simulink model "six_pulse_dstack_based_rectifier"  (R2026a)
settings: Solver=ode23tb  StopTime=simlength  FixedStep=Ts  MaxStep=Tc  EnableMultiTasking=on
values from neighbouring files (symbols this model uses):
  Csnubber = 0.1e-6    (= 1e-07)    [init_model.m]
  LFu_dc = 1.2e-3    (= 0.0012)    [init_model.m]
  Rgrading = 2.4e6    (= 2400000)    [init_model.m]
  RLFu_dc = 2e-4    (= 0.0002)    [init_model.m]
  Rsnubber = 1000    [init_model.m]
  Tc = Tcontrol_rect/4000    (= 5e-08)    [init_model.m]
  Tcontrol_rect = tPWM_RECT    (= 0.0002)    [init_model.m]
  Vnom_ac_adc = 400/sqrt(3)*sqrt(2)    [init_model.m]
  w_grid = f_grid*2*pi    (= 314.159265359)    [init_model.m]
undefined symbols (not defined in the file or in its folder): magnitude, rms
libraries: fl_lib x179, nesl_utility x129, diode_rr_lib x36, ee_lib x2
(part 4 of 5)

== system six_pulse_dstack_based_rectifier/six_pulse rectifier/BR2/ssc_diode_rr_bridge/D4/D11/D11 ==
  Capacitor : fl_lib/Electrical/Electrical Elements/Capacitor  c=Csnubber_m F  r=Rsnubber_m Ohm  g=0 1/Ohm  i_specify=off  i_priority=None  i=0 A  i_nominal_specify=off  i_nominal_value=1  i_nominal_unit=A  v_specify=off  v_priority=None  v=0 V  v_nominal_specify=off  v_nominal_value=1  v_nominal_unit=V  vc_specify=off  vc_priority=High  vc=0 V  vc_nominal_specify=off  vc_nominal_value=1  vc_nominal_unit=V
  Current Sensor : fl_lib/Electrical/Electrical Sensors/Current Sensor
  Current Sensor1 : fl_lib/Electrical/Electrical Sensors/Current Sensor
  PS-Simulink Converter : nesl_utility/PS-Simulink Converter  PhysicalDomain=network_engine_domain  SubClassName=ps_output  LeftPortType=input  RightPortType=output  PseudoPeriodic=off  Frequencies=[]  VectorFormat=1-D array  Unit=A  AffineConversion=off
  PS-Simulink Converter1 : nesl_utility/PS-Simulink Converter  PhysicalDomain=network_engine_domain  SubClassName=ps_output  LeftPortType=input  RightPortType=output  PseudoPeriodic=off  Frequencies=[]  VectorFormat=1-D array  Unit=V  AffineConversion=off
  PS-Simulink Converter2 : nesl_utility/PS-Simulink Converter  PhysicalDomain=network_engine_domain  SubClassName=ps_output  LeftPortType=input  RightPortType=output  PseudoPeriodic=off  Frequencies=[]  VectorFormat=1-D array  Unit=A  AffineConversion=off
  RR Diode (Lauritzen-Ma) : diode_rr_lib/RR Diode (Lauritzen-Ma)  Is=5e-9 A  N=2  Vt=26e-3 V  tau=350e-9 s  TM=60e-9 s  Rs=0.5e-3 Ohm  Cj0=10e-9 F  Vjp=0.7 V  mg=0.5  FC=0.5  dsm=10e-3 V  i_specify=off  i_priority=None  i=0 A  i_nominal_specify=off  i_nominal_value=1  i_nominal_unit=A  v_specify=off  v_priority=None  v=0 V  v_nominal_specify=off  v_nominal_value=1  v_nominal_unit=V  vj_specify=off  vj_priority=None  vj=0 V  vj_nominal_specify=off  vj_nominal_value=1  vj_nominal_unit=V  qE_specify=off  qE_priority=None  qE=0 C  qE_nominal_specify=off  qE_nominal_value=1e-4  qE_nominal_unit=C  qM_specify=off  qM_priority=High  qM=0 C  qM_nominal_specify=off  qM_nominal_value=1e-4  qM_nominal_unit=C  qj_specify=off  qj_priority=None  qj=0 C  qj_nominal_specify=off  qj_nominal_value=1e-5  qj_nominal_unit=C
  Voltage Sensor : fl_lib/Electrical/Electrical Sensors/Voltage Sensor
  K : PMIOPort  Side=Left
  A : PMIOPort  Port=2  Side=Right
  tag scope: D11_Id=scoped, D11_Ud=scoped, RC11_Id=scoped
  wires:
  PS-Simulink Converter/1 -> [D11_Id]
  PS-Simulink Converter2/1 -> [RC11_Id]
  PS-Simulink Converter1/1 -> [D11_Ud]
  connections:
  Voltage Sensor/RConn2 -- K/RConn1 -- Capacitor/LConn1 -- RR Diode (Lauritzen-Ma)/RConn1
  PS-Simulink Converter1/LConn1 -- Voltage Sensor/RConn1
  PS-Simulink Converter/LConn1 -- Current Sensor/RConn1
  Current Sensor1/RConn2 -- Capacitor/RConn1
  Voltage Sensor/LConn1 -- Current Sensor1/LConn1 -- Current Sensor/RConn2 -- RR Diode (Lauritzen-Ma)/LConn1
  PS-Simulink Converter2/LConn1 -- Current Sensor1/RConn1
  A/RConn1 -- Current Sensor/LConn1

== system six_pulse_dstack_based_rectifier/six_pulse rectifier/BR2/ssc_diode_rr_bridge/D4/D12/D12 ==
  Capacitor : fl_lib/Electrical/Electrical Elements/Capacitor  c=Csnubber_m F  r=Rsnubber_m Ohm  g=0 1/Ohm  i_specify=off  i_priority=None  i=0 A  i_nominal_specify=off  i_nominal_value=1  i_nominal_unit=A  v_specify=off  v_priority=None  v=0 V  v_nominal_specify=off  v_nominal_value=1  v_nominal_unit=V  vc_specify=off  vc_priority=High  vc=0 V  vc_nominal_specify=off  vc_nominal_value=1  vc_nominal_unit=V
  Current Sensor : fl_lib/Electrical/Electrical Sensors/Current Sensor
  Current Sensor1 : fl_lib/Electrical/Electrical Sensors/Current Sensor
  PS-Simulink Converter : nesl_utility/PS-Simulink Converter  PhysicalDomain=network_engine_domain  SubClassName=ps_output  LeftPortType=input  RightPortType=output  PseudoPeriodic=off  Frequencies=[]  VectorFormat=1-D array  Unit=A  AffineConversion=off
  PS-Simulink Converter1 : nesl_utility/PS-Simulink Converter  PhysicalDomain=network_engine_domain  SubClassName=ps_output  LeftPortType=input  RightPortType=output  PseudoPeriodic=off  Frequencies=[]  VectorFormat=1-D array  Unit=V  AffineConversion=off
  PS-Simulink Converter2 : nesl_utility/PS-Simulink Converter  PhysicalDomain=network_engine_domain  SubClassName=ps_output  LeftPortType=input  RightPortType=output  PseudoPeriodic=off  Frequencies=[]  VectorFormat=1-D array  Unit=A  AffineConversion=off
  RR Diode (Lauritzen-Ma) : diode_rr_lib/RR Diode (Lauritzen-Ma)  Is=5e-9 A  N=2  Vt=26e-3 V  tau=350e-9 s  TM=60e-9 s  Rs=0.5e-3 Ohm  Cj0=10e-9 F  Vjp=0.7 V  mg=0.5  FC=0.5  dsm=10e-3 V  i_specify=off  i_priority=None  i=0 A  i_nominal_specify=off  i_nominal_value=1  i_nominal_unit=A  v_specify=off  v_priority=None  v=0 V  v_nominal_specify=off  v_nominal_value=1  v_nominal_unit=V  vj_specify=off  vj_priority=None  vj=0 V  vj_nominal_specify=off  vj_nominal_value=1  vj_nominal_unit=V  qE_specify=off  qE_priority=None  qE=0 C  qE_nominal_specify=off  qE_nominal_value=1e-4  qE_nominal_unit=C  qM_specify=off  qM_priority=High  qM=0 C  qM_nominal_specify=off  qM_nominal_value=1e-4  qM_nominal_unit=C  qj_specify=off  qj_priority=None  qj=0 C  qj_nominal_specify=off  qj_nominal_value=1e-5  qj_nominal_unit=C
  Voltage Sensor : fl_lib/Electrical/Electrical Sensors/Voltage Sensor
  K : PMIOPort  Side=Left
  A : PMIOPort  Port=2  Side=Right
  tag scope: D12_Id=scoped, D12_Ud=scoped, RC12_Id=scoped
  wires:
  PS-Simulink Converter1/1 -> [D12_Ud]
  PS-Simulink Converter2/1 -> [RC12_Id]
  PS-Simulink Converter/1 -> [D12_Id]
  connections:
  A/RConn1 -- Current Sensor/LConn1
  PS-Simulink Converter2/LConn1 -- Current Sensor1/RConn1
  RR Diode (Lauritzen-Ma)/LConn1 -- Current Sensor/RConn2 -- Current Sensor1/LConn1 -- Voltage Sensor/LConn1
  Current Sensor1/RConn2 -- Capacitor/RConn1
  PS-Simulink Converter/LConn1 -- Current Sensor/RConn1
  PS-Simulink Converter1/LConn1 -- Voltage Sensor/RConn1
  RR Diode (Lauritzen-Ma)/RConn1 -- Capacitor/LConn1 -- Voltage Sensor/RConn2 -- K/RConn1

== system six_pulse_dstack_based_rectifier/six_pulse rectifier/BR2/ssc_diode_rr_bridge/D4/D13/D13 ==
  Capacitor : fl_lib/Electrical/Electrical Elements/Capacitor  c=Csnubber_m F  r=Rsnubber_m Ohm  g=0 1/Ohm  i_specify=off  i_priority=None  i=0 A  i_nominal_specify=off  i_nominal_value=1  i_nominal_unit=A  v_specify=off  v_priority=None  v=0 V  v_nominal_specify=off  v_nominal_value=1  v_nominal_unit=V  vc_specify=off  vc_priority=High  vc=0 V  vc_nominal_specify=off  vc_nominal_value=1  vc_nominal_unit=V
  Current Sensor : fl_lib/Electrical/Electrical Sensors/Current Sensor
  Current Sensor1 : fl_lib/Electrical/Electrical Sensors/Current Sensor
  PS-Simulink Converter : nesl_utility/PS-Simulink Converter  PhysicalDomain=network_engine_domain  SubClassName=ps_output  LeftPortType=input  RightPortType=output  PseudoPeriodic=off  Frequencies=[]  VectorFormat=1-D array  Unit=A  AffineConversion=off
  PS-Simulink Converter1 : nesl_utility/PS-Simulink Converter  PhysicalDomain=network_engine_domain  SubClassName=ps_output  LeftPortType=input  RightPortType=output  PseudoPeriodic=off  Frequencies=[]  VectorFormat=1-D array  Unit=V  AffineConversion=off
  PS-Simulink Converter2 : nesl_utility/PS-Simulink Converter  PhysicalDomain=network_engine_domain  SubClassName=ps_output  LeftPortType=input  RightPortType=output  PseudoPeriodic=off  Frequencies=[]  VectorFormat=1-D array  Unit=A  AffineConversion=off
  RR Diode (Lauritzen-Ma) : diode_rr_lib/RR Diode (Lauritzen-Ma)  Is=5e-9 A  N=2  Vt=26e-3 V  tau=350e-9 s  TM=60e-9 s  Rs=0.5e-3 Ohm  Cj0=10e-9 F  Vjp=0.7 V  mg=0.5  FC=0.5  dsm=10e-3 V  i_specify=off  i_priority=None  i=0 A  i_nominal_specify=off  i_nominal_value=1  i_nominal_unit=A  v_specify=off  v_priority=None  v=0 V  v_nominal_specify=off  v_nominal_value=1  v_nominal_unit=V  vj_specify=off  vj_priority=None  vj=0 V  vj_nominal_specify=off  vj_nominal_value=1  vj_nominal_unit=V  qE_specify=off  qE_priority=None  qE=0 C  qE_nominal_specify=off  qE_nominal_value=1e-4  qE_nominal_unit=C  qM_specify=off  qM_priority=High  qM=0 C  qM_nominal_specify=off  qM_nominal_value=1e-4  qM_nominal_unit=C  qj_specify=off  qj_priority=None  qj=0 C  qj_nominal_specify=off  qj_nominal_value=1e-5  qj_nominal_unit=C
  Voltage Sensor : fl_lib/Electrical/Electrical Sensors/Voltage Sensor
  K : PMIOPort  Side=Left
  A : PMIOPort  Port=2  Side=Right
  tag scope: D13_Id=scoped, D13_Ud=scoped, RC13_Id=scoped
  wires:
  PS-Simulink Converter/1 -> [D13_Id]
  PS-Simulink Converter2/1 -> [RC13_Id]
  PS-Simulink Converter1/1 -> [D13_Ud]
  connections:
  K/RConn1 -- Voltage Sensor/RConn2 -- Capacitor/LConn1 -- RR Diode (Lauritzen-Ma)/RConn1
  PS-Simulink Converter1/LConn1 -- Voltage Sensor/RConn1
  PS-Simulink Converter/LConn1 -- Current Sensor/RConn1
  Current Sensor1/RConn2 -- Capacitor/RConn1
  Voltage Sensor/LConn1 -- Current Sensor1/LConn1 -- Current Sensor/RConn2 -- RR Diode (Lauritzen-Ma)/LConn1
  PS-Simulink Converter2/LConn1 -- Current Sensor1/RConn1
  A/RConn1 -- Current Sensor/LConn1

== system six_pulse_dstack_based_rectifier/six_pulse rectifier/BR2/ssc_diode_rr_bridge/D4/D14/D14 ==
  Capacitor : fl_lib/Electrical/Electrical Elements/Capacitor  c=Csnubber_m F  r=Rsnubber_m Ohm  g=0 1/Ohm  i_specify=off  i_priority=None  i=0 A  i_nominal_specify=off  i_nominal_value=1  i_nominal_unit=A  v_specify=off  v_priority=None  v=0 V  v_nominal_specify=off  v_nominal_value=1  v_nominal_unit=V  vc_specify=off  vc_priority=High  vc=0 V  vc_nominal_specify=off  vc_nominal_value=1  vc_nominal_unit=V
  Current Sensor : fl_lib/Electrical/Electrical Sensors/Current Sensor
  Current Sensor1 : fl_lib/Electrical/Electrical Sensors/Current Sensor
  PS-Simulink Converter : nesl_utility/PS-Simulink Converter  PhysicalDomain=network_engine_domain  SubClassName=ps_output  LeftPortType=input  RightPortType=output  PseudoPeriodic=off  Frequencies=[]  VectorFormat=1-D array  Unit=A  AffineConversion=off
  PS-Simulink Converter1 : nesl_utility/PS-Simulink Converter  PhysicalDomain=network_engine_domain  SubClassName=ps_output  LeftPortType=input  RightPortType=output  PseudoPeriodic=off  Frequencies=[]  VectorFormat=1-D array  Unit=V  AffineConversion=off
  PS-Simulink Converter2 : nesl_utility/PS-Simulink Converter  PhysicalDomain=network_engine_domain  SubClassName=ps_output  LeftPortType=input  RightPortType=output  PseudoPeriodic=off  Frequencies=[]  VectorFormat=1-D array  Unit=A  AffineConversion=off
  RR Diode (Lauritzen-Ma) : diode_rr_lib/RR Diode (Lauritzen-Ma)  Is=5e-9 A  N=2  Vt=26e-3 V  tau=350e-9 s  TM=60e-9 s  Rs=0.5e-3 Ohm  Cj0=10e-9 F  Vjp=0.7 V  mg=0.5  FC=0.5  dsm=10e-3 V  i_specify=off  i_priority=None  i=0 A  i_nominal_specify=off  i_nominal_value=1  i_nominal_unit=A  v_specify=off  v_priority=None  v=0 V  v_nominal_specify=off  v_nominal_value=1  v_nominal_unit=V  vj_specify=off  vj_priority=None  vj=0 V  vj_nominal_specify=off  vj_nominal_value=1  vj_nominal_unit=V  qE_specify=off  qE_priority=None  qE=0 C  qE_nominal_specify=off  qE_nominal_value=1e-4  qE_nominal_unit=C  qM_specify=off  qM_priority=High  qM=0 C  qM_nominal_specify=off  qM_nominal_value=1e-4  qM_nominal_unit=C  qj_specify=off  qj_priority=None  qj=0 C  qj_nominal_specify=off  qj_nominal_value=1e-5  qj_nominal_unit=C
  Voltage Sensor : fl_lib/Electrical/Electrical Sensors/Voltage Sensor
  K : PMIOPort  Side=Left
  A : PMIOPort  Port=2  Side=Right
  tag scope: D14_Id=scoped, D14_Ud=scoped, RC14_Id=scoped
  wires:
  PS-Simulink Converter1/1 -> [D14_Ud]
  PS-Simulink Converter2/1 -> [RC14_Id]
  PS-Simulink Converter/1 -> [D14_Id]
  connections:
  A/RConn1 -- Current Sensor/LConn1
  PS-Simulink Converter2/LConn1 -- Current Sensor1/RConn1
  RR Diode (Lauritzen-Ma)/LConn1 -- Current Sensor/RConn2 -- Current Sensor1/LConn1 -- Voltage Sensor/LConn1
  Current Sensor1/RConn2 -- Capacitor/RConn1
  PS-Simulink Converter/LConn1 -- Current Sensor/RConn1
  PS-Simulink Converter1/LConn1 -- Voltage Sensor/RConn1
  RR Diode (Lauritzen-Ma)/RConn1 -- Capacitor/LConn1 -- Voltage Sensor/RConn2 -- K/RConn1

== system six_pulse_dstack_based_rectifier/six_pulse rectifier/BR2/ssc_diode_rr_bridge/D4/D15/D15 ==
  Capacitor : fl_lib/Electrical/Electrical Elements/Capacitor  c=Csnubber_m F  r=Rsnubber_m Ohm  g=0 1/Ohm  i_specify=off  i_priority=None  i=0 A  i_nominal_specify=off  i_nominal_value=1  i_nominal_unit=A  v_specify=off  v_priority=None  v=0 V  v_nominal_specify=off  v_nominal_value=1  v_nominal_unit=V  vc_specify=off  vc_priority=High  vc=0 V  vc_nominal_specify=off  vc_nominal_value=1  vc_nominal_unit=V
  Current Sensor : fl_lib/Electrical/Electrical Sensors/Current Sensor
  Current Sensor1 : fl_lib/Electrical/Electrical Sensors/Current Sensor
  PS-Simulink Converter : nesl_utility/PS-Simulink Converter  PhysicalDomain=network_engine_domain  SubClassName=ps_output  LeftPortType=input  RightPortType=output  PseudoPeriodic=off  Frequencies=[]  VectorFormat=1-D array  Unit=A  AffineConversion=off
  PS-Simulink Converter1 : nesl_utility/PS-Simulink Converter  PhysicalDomain=network_engine_domain  SubClassName=ps_output  LeftPortType=input  RightPortType=output  PseudoPeriodic=off  Frequencies=[]  VectorFormat=1-D array  Unit=V  AffineConversion=off
  PS-Simulink Converter2 : nesl_utility/PS-Simulink Converter  PhysicalDomain=network_engine_domain  SubClassName=ps_output  LeftPortType=input  RightPortType=output  PseudoPeriodic=off  Frequencies=[]  VectorFormat=1-D array  Unit=A  AffineConversion=off
  RR Diode (Lauritzen-Ma) : diode_rr_lib/RR Diode (Lauritzen-Ma)  Is=5e-9 A  N=2  Vt=26e-3 V  tau=350e-9 s  TM=60e-9 s  Rs=0.5e-3 Ohm  Cj0=10e-9 F  Vjp=0.7 V  mg=0.5  FC=0.5  dsm=10e-3 V  i_specify=off  i_priority=None  i=0 A  i_nominal_specify=off  i_nominal_value=1  i_nominal_unit=A  v_specify=off  v_priority=None  v=0 V  v_nominal_specify=off  v_nominal_value=1  v_nominal_unit=V  vj_specify=off  vj_priority=None  vj=0 V  vj_nominal_specify=off  vj_nominal_value=1  vj_nominal_unit=V  qE_specify=off  qE_priority=None  qE=0 C  qE_nominal_specify=off  qE_nominal_value=1e-4  qE_nominal_unit=C  qM_specify=off  qM_priority=High  qM=0 C  qM_nominal_specify=off  qM_nominal_value=1e-4  qM_nominal_unit=C  qj_specify=off  qj_priority=None  qj=0 C  qj_nominal_specify=off  qj_nominal_value=1e-5  qj_nominal_unit=C
  Voltage Sensor : fl_lib/Electrical/Electrical Sensors/Voltage Sensor
  K : PMIOPort  Side=Left
  A : PMIOPort  Port=2  Side=Right
  tag scope: D15_Id=scoped, D15_Ud=scoped, RC15_Id=scoped
  wires:
  PS-Simulink Converter/1 -> [D15_Id]
  PS-Simulink Converter2/1 -> [RC15_Id]
  PS-Simulink Converter1/1 -> [D15_Ud]
  connections:
  K/RConn1 -- Voltage Sensor/RConn2 -- Capacitor/LConn1 -- RR Diode (Lauritzen-Ma)/RConn1
  PS-Simulink Converter1/LConn1 -- Voltage Sensor/RConn1
  PS-Simulink Converter/LConn1 -- Current Sensor/RConn1
  Current Sensor1/RConn2 -- Capacitor/RConn1
  Voltage Sensor/LConn1 -- Current Sensor1/LConn1 -- Current Sensor/RConn2 -- RR Diode (Lauritzen-Ma)/LConn1
  PS-Simulink Converter2/LConn1 -- Current Sensor1/RConn1
  A/RConn1 -- Current Sensor/LConn1

== system six_pulse_dstack_based_rectifier/six_pulse rectifier/BR2/ssc_diode_rr_bridge/D4/D16/D16 ==
  Capacitor : fl_lib/Electrical/Electrical Elements/Capacitor  c=Csnubber_m F  r=Rsnubber_m Ohm  g=0 1/Ohm  i_specify=off  i_priority=None  i=0 A  i_nominal_specify=off  i_nominal_value=1  i_nominal_unit=A  v_specify=off  v_priority=None  v=0 V  v_nominal_specify=off  v_nominal_value=1  v_nominal_unit=V  vc_specify=off  vc_priority=High  vc=0 V  vc_nominal_specify=off  vc_nominal_value=1  vc_nominal_unit=V
  Current Sensor : fl_lib/Electrical/Electrical Sensors/Current Sensor
  Current Sensor1 : fl_lib/Electrical/Electrical Sensors/Current Sensor
  PS-Simulink Converter : nesl_utility/PS-Simulink Converter  PhysicalDomain=network_engine_domain  SubClassName=ps_output  LeftPortType=input  RightPortType=output  PseudoPeriodic=off  Frequencies=[]  VectorFormat=1-D array  Unit=A  AffineConversion=off
  PS-Simulink Converter1 : nesl_utility/PS-Simulink Converter  PhysicalDomain=network_engine_domain  SubClassName=ps_output  LeftPortType=input  RightPortType=output  PseudoPeriodic=off  Frequencies=[]  VectorFormat=1-D array  Unit=V  AffineConversion=off
  PS-Simulink Converter2 : nesl_utility/PS-Simulink Converter  PhysicalDomain=network_engine_domain  SubClassName=ps_output  LeftPortType=input  RightPortType=output  PseudoPeriodic=off  Frequencies=[]  VectorFormat=1-D array  Unit=A  AffineConversion=off
  RR Diode (Lauritzen-Ma) : diode_rr_lib/RR Diode (Lauritzen-Ma)  Is=5e-9 A  N=2  Vt=26e-3 V  tau=350e-9 s  TM=60e-9 s  Rs=0.5e-3 Ohm  Cj0=10e-9 F  Vjp=0.7 V  mg=0.5  FC=0.5  dsm=10e-3 V  i_specify=off  i_priority=None  i=0 A  i_nominal_specify=off  i_nominal_value=1  i_nominal_unit=A  v_specify=off  v_priority=None  v=0 V  v_nominal_specify=off  v_nominal_value=1  v_nominal_unit=V  vj_specify=off  vj_priority=None  vj=0 V  vj_nominal_specify=off  vj_nominal_value=1  vj_nominal_unit=V  qE_specify=off  qE_priority=None  qE=0 C  qE_nominal_specify=off  qE_nominal_value=1e-4  qE_nominal_unit=C  qM_specify=off  qM_priority=High  qM=0 C  qM_nominal_specify=off  qM_nominal_value=1e-4  qM_nominal_unit=C  qj_specify=off  qj_priority=None  qj=0 C  qj_nominal_specify=off  qj_nominal_value=1e-5  qj_nominal_unit=C
  Voltage Sensor : fl_lib/Electrical/Electrical Sensors/Voltage Sensor
  K : PMIOPort  Side=Left
  A : PMIOPort  Port=2  Side=Right
  tag scope: D16_Id=scoped, D16_Ud=scoped, RC16_Id=scoped
  wires:
  PS-Simulink Converter1/1 -> [D16_Ud]
  PS-Simulink Converter2/1 -> [RC16_Id]
  PS-Simulink Converter/1 -> [D16_Id]
  connections:
  A/RConn1 -- Current Sensor/LConn1
  PS-Simulink Converter2/LConn1 -- Current Sensor1/RConn1
  RR Diode (Lauritzen-Ma)/LConn1 -- Current Sensor/RConn2 -- Current Sensor1/LConn1 -- Voltage Sensor/LConn1
  Current Sensor1/RConn2 -- Capacitor/RConn1
  PS-Simulink Converter/LConn1 -- Current Sensor/RConn1
  PS-Simulink Converter1/LConn1 -- Voltage Sensor/RConn1
  RR Diode (Lauritzen-Ma)/RConn1 -- Capacitor/LConn1 -- Voltage Sensor/RConn2 -- K/RConn1

== system six_pulse_dstack_based_rectifier/six_pulse rectifier/BR2/ssc_diode_rr_bridge/D5/D11/D11 ==
  Capacitor : fl_lib/Electrical/Electrical Elements/Capacitor  c=Csnubber_m F  r=Rsnubber_m Ohm  g=0 1/Ohm  i_specify=off  i_priority=None  i=0 A  i_nominal_specify=off  i_nominal_value=1  i_nominal_unit=A  v_specify=off  v_priority=None  v=0 V  v_nominal_specify=off  v_nominal_value=1  v_nominal_unit=V  vc_specify=off  vc_priority=High  vc=0 V  vc_nominal_specify=off  vc_nominal_value=1  vc_nominal_unit=V
  Current Sensor : fl_lib/Electrical/Electrical Sensors/Current Sensor
  Current Sensor1 : fl_lib/Electrical/Electrical Sensors/Current Sensor
  PS-Simulink Converter : nesl_utility/PS-Simulink Converter  PhysicalDomain=network_engine_domain  SubClassName=ps_output  LeftPortType=input  RightPortType=output  PseudoPeriodic=off  Frequencies=[]  VectorFormat=1-D array  Unit=A  AffineConversion=off
  PS-Simulink Converter1 : nesl_utility/PS-Simulink Converter  PhysicalDomain=network_engine_domain  SubClassName=ps_output  LeftPortType=input  RightPortType=output  PseudoPeriodic=off  Frequencies=[]  VectorFormat=1-D array  Unit=V  AffineConversion=off
  PS-Simulink Converter2 : nesl_utility/PS-Simulink Converter  PhysicalDomain=network_engine_domain  SubClassName=ps_output  LeftPortType=input  RightPortType=output  PseudoPeriodic=off  Frequencies=[]  VectorFormat=1-D array  Unit=A  AffineConversion=off
  RR Diode (Lauritzen-Ma) : diode_rr_lib/RR Diode (Lauritzen-Ma)  Is=5e-9 A  N=2  Vt=26e-3 V  tau=350e-9 s  TM=60e-9 s  Rs=0.5e-3 Ohm  Cj0=10e-9 F  Vjp=0.7 V  mg=0.5  FC=0.5  dsm=10e-3 V  i_specify=off  i_priority=None  i=0 A  i_nominal_specify=off  i_nominal_value=1  i_nominal_unit=A  v_specify=off  v_priority=None  v=0 V  v_nominal_specify=off  v_nominal_value=1  v_nominal_unit=V  vj_specify=off  vj_priority=None  vj=0 V  vj_nominal_specify=off  vj_nominal_value=1  vj_nominal_unit=V  qE_specify=off  qE_priority=None  qE=0 C  qE_nominal_specify=off  qE_nominal_value=1e-4  qE_nominal_unit=C  qM_specify=off  qM_priority=High  qM=0 C  qM_nominal_specify=off  qM_nominal_value=1e-4  qM_nominal_unit=C  qj_specify=off  qj_priority=None  qj=0 C  qj_nominal_specify=off  qj_nominal_value=1e-5  qj_nominal_unit=C
  Voltage Sensor : fl_lib/Electrical/Electrical Sensors/Voltage Sensor
  K : PMIOPort  Side=Left
  A : PMIOPort  Port=2  Side=Right
  tag scope: D11_Id=scoped, D11_Ud=scoped, RC11_Id=scoped
  wires:
  PS-Simulink Converter/1 -> [D11_Id]
  PS-Simulink Converter2/1 -> [RC11_Id]
  PS-Simulink Converter1/1 -> [D11_Ud]
  connections:
  Voltage Sensor/RConn2 -- K/RConn1 -- Capacitor/LConn1 -- RR Diode (Lauritzen-Ma)/RConn1
  PS-Simulink Converter1/LConn1 -- Voltage Sensor/RConn1
  PS-Simulink Converter/LConn1 -- Current Sensor/RConn1
  Current Sensor1/RConn2 -- Capacitor/RConn1
  Voltage Sensor/LConn1 -- Current Sensor1/LConn1 -- Current Sensor/RConn2 -- RR Diode (Lauritzen-Ma)/LConn1
  PS-Simulink Converter2/LConn1 -- Current Sensor1/RConn1
  A/RConn1 -- Current Sensor/LConn1

== system six_pulse_dstack_based_rectifier/six_pulse rectifier/BR2/ssc_diode_rr_bridge/D5/D12/D12 ==
  Capacitor : fl_lib/Electrical/Electrical Elements/Capacitor  c=Csnubber_m F  r=Rsnubber_m Ohm  g=0 1/Ohm  i_specify=off  i_priority=None  i=0 A  i_nominal_specify=off  i_nominal_value=1  i_nominal_unit=A  v_specify=off  v_priority=None  v=0 V  v_nominal_specify=off  v_nominal_value=1  v_nominal_unit=V  vc_specify=off  vc_priority=High  vc=0 V  vc_nominal_specify=off  vc_nominal_value=1  vc_nominal_unit=V
  Current Sensor : fl_lib/Electrical/Electrical Sensors/Current Sensor
  Current Sensor1 : fl_lib/Electrical/Electrical Sensors/Current Sensor
  PS-Simulink Converter : nesl_utility/PS-Simulink Converter  PhysicalDomain=network_engine_domain  SubClassName=ps_output  LeftPortType=input  RightPortType=output  PseudoPeriodic=off  Frequencies=[]  VectorFormat=1-D array  Unit=A  AffineConversion=off
  PS-Simulink Converter1 : nesl_utility/PS-Simulink Converter  PhysicalDomain=network_engine_domain  SubClassName=ps_output  LeftPortType=input  RightPortType=output  PseudoPeriodic=off  Frequencies=[]  VectorFormat=1-D array  Unit=V  AffineConversion=off
  PS-Simulink Converter2 : nesl_utility/PS-Simulink Converter  PhysicalDomain=network_engine_domain  SubClassName=ps_output  LeftPortType=input  RightPortType=output  PseudoPeriodic=off  Frequencies=[]  VectorFormat=1-D array  Unit=A  AffineConversion=off
  RR Diode (Lauritzen-Ma) : diode_rr_lib/RR Diode (Lauritzen-Ma)  Is=5e-9 A  N=2  Vt=26e-3 V  tau=350e-9 s  TM=60e-9 s  Rs=0.5e-3 Ohm  Cj0=10e-9 F  Vjp=0.7 V  mg=0.5  FC=0.5  dsm=10e-3 V  i_specify=off  i_priority=None  i=0 A  i_nominal_specify=off  i_nominal_value=1  i_nominal_unit=A  v_specify=off  v_priority=None  v=0 V  v_nominal_specify=off  v_nominal_value=1  v_nominal_unit=V  vj_specify=off  vj_priority=None  vj=0 V  vj_nominal_specify=off  vj_nominal_value=1  vj_nominal_unit=V  qE_specify=off  qE_priority=None  qE=0 C  qE_nominal_specify=off  qE_nominal_value=1e-4  qE_nominal_unit=C  qM_specify=off  qM_priority=High  qM=0 C  qM_nominal_specify=off  qM_nominal_value=1e-4  qM_nominal_unit=C  qj_specify=off  qj_priority=None  qj=0 C  qj_nominal_specify=off  qj_nominal_value=1e-5  qj_nominal_unit=C
  Voltage Sensor : fl_lib/Electrical/Electrical Sensors/Voltage Sensor
  K : PMIOPort  Side=Left
  A : PMIOPort  Port=2  Side=Right
  tag scope: D12_Id=scoped, D12_Ud=scoped, RC12_Id=scoped
  wires:
  PS-Simulink Converter1/1 -> [D12_Ud]
  PS-Simulink Converter2/1 -> [RC12_Id]
  PS-Simulink Converter/1 -> [D12_Id]
  connections:
  A/RConn1 -- Current Sensor/LConn1
  PS-Simulink Converter2/LConn1 -- Current Sensor1/RConn1
  RR Diode (Lauritzen-Ma)/LConn1 -- Current Sensor/RConn2 -- Current Sensor1/LConn1 -- Voltage Sensor/LConn1
  Current Sensor1/RConn2 -- Capacitor/RConn1
  PS-Simulink Converter/LConn1 -- Current Sensor/RConn1
  PS-Simulink Converter1/LConn1 -- Voltage Sensor/RConn1
  RR Diode (Lauritzen-Ma)/RConn1 -- Capacitor/LConn1 -- Voltage Sensor/RConn2 -- K/RConn1

== system six_pulse_dstack_based_rectifier/six_pulse rectifier/BR2/ssc_diode_rr_bridge/D5/D13/D13 ==
  Capacitor : fl_lib/Electrical/Electrical Elements/Capacitor  c=Csnubber_m F  r=Rsnubber_m Ohm  g=0 1/Ohm  i_specify=off  i_priority=None  i=0 A  i_nominal_specify=off  i_nominal_value=1  i_nominal_unit=A  v_specify=off  v_priority=None  v=0 V  v_nominal_specify=off  v_nominal_value=1  v_nominal_unit=V  vc_specify=off  vc_priority=High  vc=0 V  vc_nominal_specify=off  vc_nominal_value=1  vc_nominal_unit=V
  Current Sensor : fl_lib/Electrical/Electrical Sensors/Current Sensor
  Current Sensor1 : fl_lib/Electrical/Electrical Sensors/Current Sensor
  PS-Simulink Converter : nesl_utility/PS-Simulink Converter  PhysicalDomain=network_engine_domain  SubClassName=ps_output  LeftPortType=input  RightPortType=output  PseudoPeriodic=off  Frequencies=[]  VectorFormat=1-D array  Unit=A  AffineConversion=off
  PS-Simulink Converter1 : nesl_utility/PS-Simulink Converter  PhysicalDomain=network_engine_domain  SubClassName=ps_output  LeftPortType=input  RightPortType=output  PseudoPeriodic=off  Frequencies=[]  VectorFormat=1-D array  Unit=V  AffineConversion=off
  PS-Simulink Converter2 : nesl_utility/PS-Simulink Converter  PhysicalDomain=network_engine_domain  SubClassName=ps_output  LeftPortType=input  RightPortType=output  PseudoPeriodic=off  Frequencies=[]  VectorFormat=1-D array  Unit=A  AffineConversion=off
  RR Diode (Lauritzen-Ma) : diode_rr_lib/RR Diode (Lauritzen-Ma)  Is=5e-9 A  N=2  Vt=26e-3 V  tau=350e-9 s  TM=60e-9 s  Rs=0.5e-3 Ohm  Cj0=10e-9 F  Vjp=0.7 V  mg=0.5  FC=0.5  dsm=10e-3 V  i_specify=off  i_priority=None  i=0 A  i_nominal_specify=off  i_nominal_value=1  i_nominal_unit=A  v_specify=off  v_priority=None  v=0 V  v_nominal_specify=off  v_nominal_value=1  v_nominal_unit=V  vj_specify=off  vj_priority=None  vj=0 V  vj_nominal_specify=off  vj_nominal_value=1  vj_nominal_unit=V  qE_specify=off  qE_priority=None  qE=0 C  qE_nominal_specify=off  qE_nominal_value=1e-4  qE_nominal_unit=C  qM_specify=off  qM_priority=High  qM=0 C  qM_nominal_specify=off  qM_nominal_value=1e-4  qM_nominal_unit=C  qj_specify=off  qj_priority=None  qj=0 C  qj_nominal_specify=off  qj_nominal_value=1e-5  qj_nominal_unit=C
  Voltage Sensor : fl_lib/Electrical/Electrical Sensors/Voltage Sensor
  K : PMIOPort  Side=Left
  A : PMIOPort  Port=2  Side=Right
  tag scope: D13_Id=scoped, D13_Ud=scoped, RC13_Id=scoped
  wires:
  PS-Simulink Converter/1 -> [D13_Id]
  PS-Simulink Converter2/1 -> [RC13_Id]
  PS-Simulink Converter1/1 -> [D13_Ud]
  connections:
  K/RConn1 -- Voltage Sensor/RConn2 -- Capacitor/LConn1 -- RR Diode (Lauritzen-Ma)/RConn1
  PS-Simulink Converter1/LConn1 -- Voltage Sensor/RConn1
  PS-Simulink Converter/LConn1 -- Current Sensor/RConn1
  Current Sensor1/RConn2 -- Capacitor/RConn1
  Voltage Sensor/LConn1 -- Current Sensor1/LConn1 -- Current Sensor/RConn2 -- RR Diode (Lauritzen-Ma)/LConn1
  PS-Simulink Converter2/LConn1 -- Current Sensor1/RConn1
  A/RConn1 -- Current Sensor/LConn1

== system six_pulse_dstack_based_rectifier/six_pulse rectifier/BR2/ssc_diode_rr_bridge/D5/D14/D14 ==
  Capacitor : fl_lib/Electrical/Electrical Elements/Capacitor  c=Csnubber_m F  r=Rsnubber_m Ohm  g=0 1/Ohm  i_specify=off  i_priority=None  i=0 A  i_nominal_specify=off  i_nominal_value=1  i_nominal_unit=A  v_specify=off  v_priority=None  v=0 V  v_nominal_specify=off  v_nominal_value=1  v_nominal_unit=V  vc_specify=off  vc_priority=High  vc=0 V  vc_nominal_specify=off  vc_nominal_value=1  vc_nominal_unit=V
  Current Sensor : fl_lib/Electrical/Electrical Sensors/Current Sensor
  Current Sensor1 : fl_lib/Electrical/Electrical Sensors/Current Sensor
  PS-Simulink Converter : nesl_utility/PS-Simulink Converter  PhysicalDomain=network_engine_domain  SubClassName=ps_output  LeftPortType=input  RightPortType=output  PseudoPeriodic=off  Frequencies=[]  VectorFormat=1-D array  Unit=A  AffineConversion=off
  PS-Simulink Converter1 : nesl_utility/PS-Simulink Converter  PhysicalDomain=network_engine_domain  SubClassName=ps_output  LeftPortType=input  RightPortType=output  PseudoPeriodic=off  Frequencies=[]  VectorFormat=1-D array  Unit=V  AffineConversion=off
  PS-Simulink Converter2 : nesl_utility/PS-Simulink Converter  PhysicalDomain=network_engine_domain  SubClassName=ps_output  LeftPortType=input  RightPortType=output  PseudoPeriodic=off  Frequencies=[]  VectorFormat=1-D array  Unit=A  AffineConversion=off
  RR Diode (Lauritzen-Ma) : diode_rr_lib/RR Diode (Lauritzen-Ma)  Is=5e-9 A  N=2  Vt=26e-3 V  tau=350e-9 s  TM=60e-9 s  Rs=0.5e-3 Ohm  Cj0=10e-9 F  Vjp=0.7 V  mg=0.5  FC=0.5  dsm=10e-3 V  i_specify=off  i_priority=None  i=0 A  i_nominal_specify=off  i_nominal_value=1  i_nominal_unit=A  v_specify=off  v_priority=None  v=0 V  v_nominal_specify=off  v_nominal_value=1  v_nominal_unit=V  vj_specify=off  vj_priority=None  vj=0 V  vj_nominal_specify=off  vj_nominal_value=1  vj_nominal_unit=V  qE_specify=off  qE_priority=None  qE=0 C  qE_nominal_specify=off  qE_nominal_value=1e-4  qE_nominal_unit=C  qM_specify=off  qM_priority=High  qM=0 C  qM_nominal_specify=off  qM_nominal_value=1e-4  qM_nominal_unit=C  qj_specify=off  qj_priority=None  qj=0 C  qj_nominal_specify=off  qj_nominal_value=1e-5  qj_nominal_unit=C
  Voltage Sensor : fl_lib/Electrical/Electrical Sensors/Voltage Sensor
  K : PMIOPort  Side=Left
  A : PMIOPort  Port=2  Side=Right
  tag scope: D14_Id=scoped, D14_Ud=scoped, RC14_Id=scoped
  wires:
  PS-Simulink Converter1/1 -> [D14_Ud]
  PS-Simulink Converter2/1 -> [RC14_Id]
  PS-Simulink Converter/1 -> [D14_Id]
  connections:
  A/RConn1 -- Current Sensor/LConn1
  PS-Simulink Converter2/LConn1 -- Current Sensor1/RConn1
  RR Diode (Lauritzen-Ma)/LConn1 -- Current Sensor/RConn2 -- Current Sensor1/LConn1 -- Voltage Sensor/LConn1
  Current Sensor1/RConn2 -- Capacitor/RConn1
  PS-Simulink Converter/LConn1 -- Current Sensor/RConn1
  PS-Simulink Converter1/LConn1 -- Voltage Sensor/RConn1
  RR Diode (Lauritzen-Ma)/RConn1 -- Capacitor/LConn1 -- Voltage Sensor/RConn2 -- K/RConn1

== system six_pulse_dstack_based_rectifier/six_pulse rectifier/BR2/ssc_diode_rr_bridge/D5/D15/D15 ==
  Capacitor : fl_lib/Electrical/Electrical Elements/Capacitor  c=Csnubber_m F  r=Rsnubber_m Ohm  g=0 1/Ohm  i_specify=off  i_priority=None  i=0 A  i_nominal_specify=off  i_nominal_value=1  i_nominal_unit=A  v_specify=off  v_priority=None  v=0 V  v_nominal_specify=off  v_nominal_value=1  v_nominal_unit=V  vc_specify=off  vc_priority=High  vc=0 V  vc_nominal_specify=off  vc_nominal_value=1  vc_nominal_unit=V
  Current Sensor : fl_lib/Electrical/Electrical Sensors/Current Sensor
  Current Sensor1 : fl_lib/Electrical/Electrical Sensors/Current Sensor
  PS-Simulink Converter : nesl_utility/PS-Simulink Converter  PhysicalDomain=network_engine_domain  SubClassName=ps_output  LeftPortType=input  RightPortType=output  PseudoPeriodic=off  Frequencies=[]  VectorFormat=1-D array  Unit=A  AffineConversion=off
  PS-Simulink Converter1 : nesl_utility/PS-Simulink Converter  PhysicalDomain=network_engine_domain  SubClassName=ps_output  LeftPortType=input  RightPortType=output  PseudoPeriodic=off  Frequencies=[]  VectorFormat=1-D array  Unit=V  AffineConversion=off
  PS-Simulink Converter2 : nesl_utility/PS-Simulink Converter  PhysicalDomain=network_engine_domain  SubClassName=ps_output  LeftPortType=input  RightPortType=output  PseudoPeriodic=off  Frequencies=[]  VectorFormat=1-D array  Unit=A  AffineConversion=off
  RR Diode (Lauritzen-Ma) : diode_rr_lib/RR Diode (Lauritzen-Ma)  Is=5e-9 A  N=2  Vt=26e-3 V  tau=350e-9 s  TM=60e-9 s  Rs=0.5e-3 Ohm  Cj0=10e-9 F  Vjp=0.7 V  mg=0.5  FC=0.5  dsm=10e-3 V  i_specify=off  i_priority=None  i=0 A  i_nominal_specify=off  i_nominal_value=1  i_nominal_unit=A  v_specify=off  v_priority=None  v=0 V  v_nominal_specify=off  v_nominal_value=1  v_nominal_unit=V  vj_specify=off  vj_priority=None  vj=0 V  vj_nominal_specify=off  vj_nominal_value=1  vj_nominal_unit=V  qE_specify=off  qE_priority=None  qE=0 C  qE_nominal_specify=off  qE_nominal_value=1e-4  qE_nominal_unit=C  qM_specify=off  qM_priority=High  qM=0 C  qM_nominal_specify=off  qM_nominal_value=1e-4  qM_nominal_unit=C  qj_specify=off  qj_priority=None  qj=0 C  qj_nominal_specify=off  qj_nominal_value=1e-5  qj_nominal_unit=C
  Voltage Sensor : fl_lib/Electrical/Electrical Sensors/Voltage Sensor
  K : PMIOPort  Side=Left
  A : PMIOPort  Port=2  Side=Right
  tag scope: D15_Id=scoped, D15_Ud=scoped, RC15_Id=scoped
  wires:
  PS-Simulink Converter/1 -> [D15_Id]
  PS-Simulink Converter2/1 -> [RC15_Id]
  PS-Simulink Converter1/1 -> [D15_Ud]
  connections:
  K/RConn1 -- Voltage Sensor/RConn2 -- Capacitor/LConn1 -- RR Diode (Lauritzen-Ma)/RConn1
  PS-Simulink Converter1/LConn1 -- Voltage Sensor/RConn1
  PS-Simulink Converter/LConn1 -- Current Sensor/RConn1
  Current Sensor1/RConn2 -- Capacitor/RConn1
  Voltage Sensor/LConn1 -- Current Sensor1/LConn1 -- Current Sensor/RConn2 -- RR Diode (Lauritzen-Ma)/LConn1
  PS-Simulink Converter2/LConn1 -- Current Sensor1/RConn1
  A/RConn1 -- Current Sensor/LConn1

== system six_pulse_dstack_based_rectifier/six_pulse rectifier/BR2/ssc_diode_rr_bridge/D5/D16/D16 ==
  Capacitor : fl_lib/Electrical/Electrical Elements/Capacitor  c=Csnubber_m F  r=Rsnubber_m Ohm  g=0 1/Ohm  i_specify=off  i_priority=None  i=0 A  i_nominal_specify=off  i_nominal_value=1  i_nominal_unit=A  v_specify=off  v_priority=None  v=0 V  v_nominal_specify=off  v_nominal_value=1  v_nominal_unit=V  vc_specify=off  vc_priority=High  vc=0 V  vc_nominal_specify=off  vc_nominal_value=1  vc_nominal_unit=V
  Current Sensor : fl_lib/Electrical/Electrical Sensors/Current Sensor
  Current Sensor1 : fl_lib/Electrical/Electrical Sensors/Current Sensor
  PS-Simulink Converter : nesl_utility/PS-Simulink Converter  PhysicalDomain=network_engine_domain  SubClassName=ps_output  LeftPortType=input  RightPortType=output  PseudoPeriodic=off  Frequencies=[]  VectorFormat=1-D array  Unit=A  AffineConversion=off
  PS-Simulink Converter1 : nesl_utility/PS-Simulink Converter  PhysicalDomain=network_engine_domain  SubClassName=ps_output  LeftPortType=input  RightPortType=output  PseudoPeriodic=off  Frequencies=[]  VectorFormat=1-D array  Unit=V  AffineConversion=off
  PS-Simulink Converter2 : nesl_utility/PS-Simulink Converter  PhysicalDomain=network_engine_domain  SubClassName=ps_output  LeftPortType=input  RightPortType=output  PseudoPeriodic=off  Frequencies=[]  VectorFormat=1-D array  Unit=A  AffineConversion=off
  RR Diode (Lauritzen-Ma) : diode_rr_lib/RR Diode (Lauritzen-Ma)  Is=5e-9 A  N=2  Vt=26e-3 V  tau=350e-9 s  TM=60e-9 s  Rs=0.5e-3 Ohm  Cj0=10e-9 F  Vjp=0.7 V  mg=0.5  FC=0.5  dsm=10e-3 V  i_specify=off  i_priority=None  i=0 A  i_nominal_specify=off  i_nominal_value=1  i_nominal_unit=A  v_specify=off  v_priority=None  v=0 V  v_nominal_specify=off  v_nominal_value=1  v_nominal_unit=V  vj_specify=off  vj_priority=None  vj=0 V  vj_nominal_specify=off  vj_nominal_value=1  vj_nominal_unit=V  qE_specify=off  qE_priority=None  qE=0 C  qE_nominal_specify=off  qE_nominal_value=1e-4  qE_nominal_unit=C  qM_specify=off  qM_priority=High  qM=0 C  qM_nominal_specify=off  qM_nominal_value=1e-4  qM_nominal_unit=C  qj_specify=off  qj_priority=None  qj=0 C  qj_nominal_specify=off  qj_nominal_value=1e-5  qj_nominal_unit=C
  Voltage Sensor : fl_lib/Electrical/Electrical Sensors/Voltage Sensor
  K : PMIOPort  Side=Left
  A : PMIOPort  Port=2  Side=Right
  tag scope: D16_Id=scoped, D16_Ud=scoped, RC16_Id=scoped
  wires:
  PS-Simulink Converter1/1 -> [D16_Ud]
  PS-Simulink Converter2/1 -> [RC16_Id]
  PS-Simulink Converter/1 -> [D16_Id]
  connections:
  A/RConn1 -- Current Sensor/LConn1
  PS-Simulink Converter2/LConn1 -- Current Sensor1/RConn1
  RR Diode (Lauritzen-Ma)/LConn1 -- Current Sensor/RConn2 -- Current Sensor1/LConn1 -- Voltage Sensor/LConn1
  Current Sensor1/RConn2 -- Capacitor/RConn1
  PS-Simulink Converter/LConn1 -- Current Sensor/RConn1
  PS-Simulink Converter1/LConn1 -- Voltage Sensor/RConn1
  RR Diode (Lauritzen-Ma)/RConn1 -- Capacitor/LConn1 -- Voltage Sensor/RConn2 -- K/RConn1

== system six_pulse_dstack_based_rectifier/six_pulse rectifier/BR2/ssc_diode_rr_bridge/D6/D11/D11 ==
  Capacitor : fl_lib/Electrical/Electrical Elements/Capacitor  c=Csnubber_m F  r=Rsnubber_m Ohm  g=0 1/Ohm  i_specify=off  i_priority=None  i=0 A  i_nominal_specify=off  i_nominal_value=1  i_nominal_unit=A  v_specify=off  v_priority=None  v=0 V  v_nominal_specify=off  v_nominal_value=1  v_nominal_unit=V  vc_specify=off  vc_priority=High  vc=0 V  vc_nominal_specify=off  vc_nominal_value=1  vc_nominal_unit=V
  Current Sensor : fl_lib/Electrical/Electrical Sensors/Current Sensor
  Current Sensor1 : fl_lib/Electrical/Electrical Sensors/Current Sensor
  PS-Simulink Converter : nesl_utility/PS-Simulink Converter  PhysicalDomain=network_engine_domain  SubClassName=ps_output  LeftPortType=input  RightPortType=output  PseudoPeriodic=off  Frequencies=[]  VectorFormat=1-D array  Unit=A  AffineConversion=off
  PS-Simulink Converter1 : nesl_utility/PS-Simulink Converter  PhysicalDomain=network_engine_domain  SubClassName=ps_output  LeftPortType=input  RightPortType=output  PseudoPeriodic=off  Frequencies=[]  VectorFormat=1-D array  Unit=V  AffineConversion=off
  PS-Simulink Converter2 : nesl_utility/PS-Simulink Converter  PhysicalDomain=network_engine_domain  SubClassName=ps_output  LeftPortType=input  RightPortType=output  PseudoPeriodic=off  Frequencies=[]  VectorFormat=1-D array  Unit=A  AffineConversion=off
  RR Diode (Lauritzen-Ma) : diode_rr_lib/RR Diode (Lauritzen-Ma)  Is=5e-9 A  N=2  Vt=26e-3 V  tau=350e-9 s  TM=60e-9 s  Rs=0.5e-3 Ohm  Cj0=10e-9 F  Vjp=0.7 V  mg=0.5  FC=0.5  dsm=10e-3 V  i_specify=off  i_priority=None  i=0 A  i_nominal_specify=off  i_nominal_value=1  i_nominal_unit=A  v_specify=off  v_priority=None  v=0 V  v_nominal_specify=off  v_nominal_value=1  v_nominal_unit=V  vj_specify=off  vj_priority=None  vj=0 V  vj_nominal_specify=off  vj_nominal_value=1  vj_nominal_unit=V  qE_specify=off  qE_priority=None  qE=0 C  qE_nominal_specify=off  qE_nominal_value=1e-4  qE_nominal_unit=C  qM_specify=off  qM_priority=High  qM=0 C  qM_nominal_specify=off  qM_nominal_value=1e-4  qM_nominal_unit=C  qj_specify=off  qj_priority=None  qj=0 C  qj_nominal_specify=off  qj_nominal_value=1e-5  qj_nominal_unit=C
  Voltage Sensor : fl_lib/Electrical/Electrical Sensors/Voltage Sensor
  K : PMIOPort  Side=Left
  A : PMIOPort  Port=2  Side=Right
  tag scope: D11_Id=scoped, D11_Ud=scoped, RC11_Id=scoped
  wires:
  PS-Simulink Converter1/1 -> [D11_Ud]
  PS-Simulink Converter2/1 -> [RC11_Id]
  PS-Simulink Converter/1 -> [D11_Id]
  connections:
  A/RConn1 -- Current Sensor/LConn1
  PS-Simulink Converter2/LConn1 -- Current Sensor1/RConn1
  RR Diode (Lauritzen-Ma)/LConn1 -- Current Sensor/RConn2 -- Current Sensor1/LConn1 -- Voltage Sensor/LConn1
  Current Sensor1/RConn2 -- Capacitor/RConn1
  PS-Simulink Converter/LConn1 -- Current Sensor/RConn1
  PS-Simulink Converter1/LConn1 -- Voltage Sensor/RConn1
  RR Diode (Lauritzen-Ma)/RConn1 -- Capacitor/LConn1 -- K/RConn1 -- Voltage Sensor/RConn2

== system six_pulse_dstack_based_rectifier/six_pulse rectifier/BR2/ssc_diode_rr_bridge/D6/D12/D12 ==
  Capacitor : fl_lib/Electrical/Electrical Elements/Capacitor  c=Csnubber_m F  r=Rsnubber_m Ohm  g=0 1/Ohm  i_specify=off  i_priority=None  i=0 A  i_nominal_specify=off  i_nominal_value=1  i_nominal_unit=A  v_specify=off  v_priority=None  v=0 V  v_nominal_specify=off  v_nominal_value=1  v_nominal_unit=V  vc_specify=off  vc_priority=High  vc=0 V  vc_nominal_specify=off  vc_nominal_value=1  vc_nominal_unit=V
  Current Sensor : fl_lib/Electrical/Electrical Sensors/Current Sensor
  Current Sensor1 : fl_lib/Electrical/Electrical Sensors/Current Sensor
  PS-Simulink Converter : nesl_utility/PS-Simulink Converter  PhysicalDomain=network_engine_domain  SubClassName=ps_output  LeftPortType=input  RightPortType=output  PseudoPeriodic=off  Frequencies=[]  VectorFormat=1-D array  Unit=A  AffineConversion=off
  PS-Simulink Converter1 : nesl_utility/PS-Simulink Converter  PhysicalDomain=network_engine_domain  SubClassName=ps_output  LeftPortType=input  RightPortType=output  PseudoPeriodic=off  Frequencies=[]  VectorFormat=1-D array  Unit=V  AffineConversion=off
  PS-Simulink Converter2 : nesl_utility/PS-Simulink Converter  PhysicalDomain=network_engine_domain  SubClassName=ps_output  LeftPortType=input  RightPortType=output  PseudoPeriodic=off  Frequencies=[]  VectorFormat=1-D array  Unit=A  AffineConversion=off
  RR Diode (Lauritzen-Ma) : diode_rr_lib/RR Diode (Lauritzen-Ma)  Is=5e-9 A  N=2  Vt=26e-3 V  tau=350e-9 s  TM=60e-9 s  Rs=0.5e-3 Ohm  Cj0=10e-9 F  Vjp=0.7 V  mg=0.5  FC=0.5  dsm=10e-3 V  i_specify=off  i_priority=None  i=0 A  i_nominal_specify=off  i_nominal_value=1  i_nominal_unit=A  v_specify=off  v_priority=None  v=0 V  v_nominal_specify=off  v_nominal_value=1  v_nominal_unit=V  vj_specify=off  vj_priority=None  vj=0 V  vj_nominal_specify=off  vj_nominal_value=1  vj_nominal_unit=V  qE_specify=off  qE_priority=None  qE=0 C  qE_nominal_specify=off  qE_nominal_value=1e-4  qE_nominal_unit=C  qM_specify=off  qM_priority=High  qM=0 C  qM_nominal_specify=off  qM_nominal_value=1e-4  qM_nominal_unit=C  qj_specify=off  qj_priority=None  qj=0 C  qj_nominal_specify=off  qj_nominal_value=1e-5  qj_nominal_unit=C
  Voltage Sensor : fl_lib/Electrical/Electrical Sensors/Voltage Sensor
  K : PMIOPort  Side=Left
  A : PMIOPort  Port=2  Side=Right
  tag scope: D12_Id=scoped, D12_Ud=scoped, RC12_Id=scoped
  wires:
  PS-Simulink Converter/1 -> [D12_Id]
  PS-Simulink Converter2/1 -> [RC12_Id]
  PS-Simulink Converter1/1 -> [D12_Ud]
  connections:
  K/RConn1 -- Voltage Sensor/RConn2 -- Capacitor/LConn1 -- RR Diode (Lauritzen-Ma)/RConn1
  PS-Simulink Converter1/LConn1 -- Voltage Sensor/RConn1
  PS-Simulink Converter/LConn1 -- Current Sensor/RConn1
  Current Sensor1/RConn2 -- Capacitor/RConn1
  Voltage Sensor/LConn1 -- Current Sensor1/LConn1 -- Current Sensor/RConn2 -- RR Diode (Lauritzen-Ma)/LConn1
  PS-Simulink Converter2/LConn1 -- Current Sensor1/RConn1
  A/RConn1 -- Current Sensor/LConn1

== system six_pulse_dstack_based_rectifier/six_pulse rectifier/BR2/ssc_diode_rr_bridge/D6/D13/D13 ==
  Capacitor : fl_lib/Electrical/Electrical Elements/Capacitor  c=Csnubber_m F  r=Rsnubber_m Ohm  g=0 1/Ohm  i_specify=off  i_priority=None  i=0 A  i_nominal_specify=off  i_nominal_value=1  i_nominal_unit=A  v_specify=off  v_priority=None  v=0 V  v_nominal_specify=off  v_nominal_value=1  v_nominal_unit=V  vc_specify=off  vc_priority=High  vc=0 V  vc_nominal_specify=off  vc_nominal_value=1  vc_nominal_unit=V
  Current Sensor : fl_lib/Electrical/Electrical Sensors/Current Sensor
  Current Sensor1 : fl_lib/Electrical/Electrical Sensors/Current Sensor
  PS-Simulink Converter : nesl_utility/PS-Simulink Converter  PhysicalDomain=network_engine_domain  SubClassName=ps_output  LeftPortType=input  RightPortType=output  PseudoPeriodic=off  Frequencies=[]  VectorFormat=1-D array  Unit=A  AffineConversion=off
  PS-Simulink Converter1 : nesl_utility/PS-Simulink Converter  PhysicalDomain=network_engine_domain  SubClassName=ps_output  LeftPortType=input  RightPortType=output  PseudoPeriodic=off  Frequencies=[]  VectorFormat=1-D array  Unit=V  AffineConversion=off
  PS-Simulink Converter2 : nesl_utility/PS-Simulink Converter  PhysicalDomain=network_engine_domain  SubClassName=ps_output  LeftPortType=input  RightPortType=output  PseudoPeriodic=off  Frequencies=[]  VectorFormat=1-D array  Unit=A  AffineConversion=off
  RR Diode (Lauritzen-Ma) : diode_rr_lib/RR Diode (Lauritzen-Ma)  Is=5e-9 A  N=2  Vt=26e-3 V  tau=350e-9 s  TM=60e-9 s  Rs=0.5e-3 Ohm  Cj0=10e-9 F  Vjp=0.7 V  mg=0.5  FC=0.5  dsm=10e-3 V  i_specify=off  i_priority=None  i=0 A  i_nominal_specify=off  i_nominal_value=1  i_nominal_unit=A  v_specify=off  v_priority=None  v=0 V  v_nominal_specify=off  v_nominal_value=1  v_nominal_unit=V  vj_specify=off  vj_priority=None  vj=0 V  vj_nominal_specify=off  vj_nominal_value=1  vj_nominal_unit=V  qE_specify=off  qE_priority=None  qE=0 C  qE_nominal_specify=off  qE_nominal_value=1e-4  qE_nominal_unit=C  qM_specify=off  qM_priority=High  qM=0 C  qM_nominal_specify=off  qM_nominal_value=1e-4  qM_nominal_unit=C  qj_specify=off  qj_priority=None  qj=0 C  qj_nominal_specify=off  qj_nominal_value=1e-5  qj_nominal_unit=C
  Voltage Sensor : fl_lib/Electrical/Electrical Sensors/Voltage Sensor
  K : PMIOPort  Side=Left
  A : PMIOPort  Port=2  Side=Right
  tag scope: D13_Id=scoped, D13_Ud=scoped, RC13_Id=scoped
  wires:
  PS-Simulink Converter1/1 -> [D13_Ud]
  PS-Simulink Converter2/1 -> [RC13_Id]
  PS-Simulink Converter/1 -> [D13_Id]
  connections:
  A/RConn1 -- Current Sensor/LConn1
  PS-Simulink Converter2/LConn1 -- Current Sensor1/RConn1
  RR Diode (Lauritzen-Ma)/LConn1 -- Current Sensor/RConn2 -- Current Sensor1/LConn1 -- Voltage Sensor/LConn1
  Current Sensor1/RConn2 -- Capacitor/RConn1
  PS-Simulink Converter/LConn1 -- Current Sensor/RConn1
  PS-Simulink Converter1/LConn1 -- Voltage Sensor/RConn1
  RR Diode (Lauritzen-Ma)/RConn1 -- Capacitor/LConn1 -- Voltage Sensor/RConn2 -- K/RConn1

== system six_pulse_dstack_based_rectifier/six_pulse rectifier/BR2/ssc_diode_rr_bridge/D6/D14/D14 ==
  Capacitor : fl_lib/Electrical/Electrical Elements/Capacitor  c=Csnubber_m F  r=Rsnubber_m Ohm  g=0 1/Ohm  i_specify=off  i_priority=None  i=0 A  i_nominal_specify=off  i_nominal_value=1  i_nominal_unit=A  v_specify=off  v_priority=None  v=0 V  v_nominal_specify=off  v_nominal_value=1  v_nominal_unit=V  vc_specify=off  vc_priority=High  vc=0 V  vc_nominal_specify=off  vc_nominal_value=1  vc_nominal_unit=V
  Current Sensor : fl_lib/Electrical/Electrical Sensors/Current Sensor
  Current Sensor1 : fl_lib/Electrical/Electrical Sensors/Current Sensor
  PS-Simulink Converter : nesl_utility/PS-Simulink Converter  PhysicalDomain=network_engine_domain  SubClassName=ps_output  LeftPortType=input  RightPortType=output  PseudoPeriodic=off  Frequencies=[]  VectorFormat=1-D array  Unit=A  AffineConversion=off
  PS-Simulink Converter1 : nesl_utility/PS-Simulink Converter  PhysicalDomain=network_engine_domain  SubClassName=ps_output  LeftPortType=input  RightPortType=output  PseudoPeriodic=off  Frequencies=[]  VectorFormat=1-D array  Unit=V  AffineConversion=off
  PS-Simulink Converter2 : nesl_utility/PS-Simulink Converter  PhysicalDomain=network_engine_domain  SubClassName=ps_output  LeftPortType=input  RightPortType=output  PseudoPeriodic=off  Frequencies=[]  VectorFormat=1-D array  Unit=A  AffineConversion=off
  RR Diode (Lauritzen-Ma) : diode_rr_lib/RR Diode (Lauritzen-Ma)  Is=5e-9 A  N=2  Vt=26e-3 V  tau=350e-9 s  TM=60e-9 s  Rs=0.5e-3 Ohm  Cj0=10e-9 F  Vjp=0.7 V  mg=0.5  FC=0.5  dsm=10e-3 V  i_specify=off  i_priority=None  i=0 A  i_nominal_specify=off  i_nominal_value=1  i_nominal_unit=A  v_specify=off  v_priority=None  v=0 V  v_nominal_specify=off  v_nominal_value=1  v_nominal_unit=V  vj_specify=off  vj_priority=None  vj=0 V  vj_nominal_specify=off  vj_nominal_value=1  vj_nominal_unit=V  qE_specify=off  qE_priority=None  qE=0 C  qE_nominal_specify=off  qE_nominal_value=1e-4  qE_nominal_unit=C  qM_specify=off  qM_priority=High  qM=0 C  qM_nominal_specify=off  qM_nominal_value=1e-4  qM_nominal_unit=C  qj_specify=off  qj_priority=None  qj=0 C  qj_nominal_specify=off  qj_nominal_value=1e-5  qj_nominal_unit=C
  Voltage Sensor : fl_lib/Electrical/Electrical Sensors/Voltage Sensor
  K : PMIOPort  Side=Left
  A : PMIOPort  Port=2  Side=Right
  tag scope: D14_Id=scoped, D14_Ud=scoped, RC14_Id=scoped
  wires:
  PS-Simulink Converter/1 -> [D14_Id]
  PS-Simulink Converter2/1 -> [RC14_Id]
  PS-Simulink Converter1/1 -> [D14_Ud]
  connections:
  K/RConn1 -- Voltage Sensor/RConn2 -- Capacitor/LConn1 -- RR Diode (Lauritzen-Ma)/RConn1
  PS-Simulink Converter1/LConn1 -- Voltage Sensor/RConn1
  PS-Simulink Converter/LConn1 -- Current Sensor/RConn1
  Current Sensor1/RConn2 -- Capacitor/RConn1
  Voltage Sensor/LConn1 -- Current Sensor1/LConn1 -- Current Sensor/RConn2 -- RR Diode (Lauritzen-Ma)/LConn1
  PS-Simulink Converter2/LConn1 -- Current Sensor1/RConn1
  A/RConn1 -- Current Sensor/LConn1
